simulink model "Hexapod_PD"  (R2026a)
settings: Solver=daessc  StopTime=ref.t(end)  FixedStep=2e-5
InitFcn:
  | startup
model workspace: external: MATLAB File Hexapod_DataFile.m (data not in the file)
undefined symbols (not defined in the file or in its folder): ref, robot, smiData, vc, X, Y, Z
libraries: sm_lib x805, nesl_utility x43
(part 9 of 15)

== system Hexapod_PD/Spherical Joints/MotorRotor_a_4_RIGID ==
  MotorRotor_1_RIGID : Subsystem
  ReferenceFrame : sm_lib/Frames and Transforms/Reference Frame
  ServoArm_1_RIGID : Subsystem
  Transform : sm_lib/Frames and Transforms/Rigid Transform  RotationMethod=ArbitraryAxis  FollAlignAxisA=+X  BaseAlignAxisA=+Y  FollAlignAxisB=+Y  BaseAlignAxisB=+Z  RotationStandardAxis=+Z  RotationAngle=smiData.RigidTransform(22).angle  RotationAngleUnits=rad  RotationArbitraryAxis=smiData.RigidTransform(22).axis  RotationSequenceAxes=FollowerAxes  RotationSequence=XYX  RotationSequenceAngles=[0 0 0]  RotationSequenceAnglesUnits=deg  RotationMatrix=[1 0 0;0 1 0;0 0 1]  Quaternion=[1 0 0 0]  TranslationMethod=Cartesian  TranslationCartesianOffset=smiData.RigidTransform(22).translation  TranslationCartesianOffsetUnits=mm  TranslationStandardAxis=+Z  TranslationStandardOffset=0  TranslationStandardOffsetUnits=m  TranslationROffset=0  TranslationROffsetUnits=m  TranslationThetaOffset=0  TranslationThetaOffsetUnits=deg  TranslationZOffset=0  TranslationZOffsetUnits=m
  Transform1 : sm_lib/Frames and Transforms/Rigid Transform  RotationMethod=ArbitraryAxis  FollAlignAxisA=+X  BaseAlignAxisA=+Y  FollAlignAxisB=+Y  BaseAlignAxisB=+Z  RotationStandardAxis=+Z  RotationAngle=smiData.RigidTransform(23).angle  RotationAngleUnits=rad  RotationArbitraryAxis=smiData.RigidTransform(23).axis  RotationSequenceAxes=FollowerAxes  RotationSequence=XYX  RotationSequenceAngles=[0 0 0]  RotationSequenceAnglesUnits=deg  RotationMatrix=[1 0 0;0 1 0;0 0 1]  Quaternion=[1 0 0 0]  TranslationMethod=Cartesian  TranslationCartesianOffset=smiData.RigidTransform(23).translation  TranslationCartesianOffsetUnits=mm  TranslationStandardAxis=+Z  TranslationStandardOffset=0  TranslationStandardOffsetUnits=m  TranslationROffset=0  TranslationROffsetUnits=m  TranslationThetaOffset=0  TranslationThetaOffsetUnits=deg  TranslationZOffset=0  TranslationZOffsetUnits=m
  Transform10 : sm_lib/Frames and Transforms/Rigid Transform  RotationMethod=ArbitraryAxis  FollAlignAxisA=+X  BaseAlignAxisA=+Y  FollAlignAxisB=+Y  BaseAlignAxisB=+Z  RotationStandardAxis=+Z  RotationAngle=smiData.RigidTransform(269).angle  RotationAngleUnits=rad  RotationArbitraryAxis=smiData.RigidTransform(269).axis  RotationSequenceAxes=FollowerAxes  RotationSequence=XYX  RotationSequenceAngles=[0 0 0]  RotationSequenceAnglesUnits=deg  RotationMatrix=[1 0 0;0 1 0;0 0 1]  Quaternion=[1 0 0 0]  TranslationMethod=Cartesian  TranslationCartesianOffset=smiData.RigidTransform(269).translation  TranslationCartesianOffsetUnits=mm  TranslationStandardAxis=+Z  TranslationStandardOffset=0  TranslationStandardOffsetUnits=m  TranslationROffset=0  TranslationROffsetUnits=m  TranslationThetaOffset=0  TranslationThetaOffsetUnits=deg  TranslationZOffset=0  TranslationZOffsetUnits=m
  Transform11 : sm_lib/Frames and Transforms/Rigid Transform  RotationMethod=ArbitraryAxis  FollAlignAxisA=+X  BaseAlignAxisA=+Y  FollAlignAxisB=+Y  BaseAlignAxisB=+Z  RotationStandardAxis=+Z  RotationAngle=smiData.RigidTransform(270).angle  RotationAngleUnits=rad  RotationArbitraryAxis=smiData.RigidTransform(270).axis  RotationSequenceAxes=FollowerAxes  RotationSequence=XYX  RotationSequenceAngles=[0 0 0]  RotationSequenceAnglesUnits=deg  RotationMatrix=[1 0 0;0 1 0;0 0 1]  Quaternion=[1 0 0 0]  TranslationMethod=Cartesian  TranslationCartesianOffset=smiData.RigidTransform(270).translation  TranslationCartesianOffsetUnits=mm  TranslationStandardAxis=+Z  TranslationStandardOffset=0  TranslationStandardOffsetUnits=m  TranslationROffset=0  TranslationROffsetUnits=m  TranslationThetaOffset=0  TranslationThetaOffsetUnits=deg  TranslationZOffset=0  TranslationZOffsetUnits=m
  Transform2 : sm_lib/Frames and Transforms/Rigid Transform  RotationMethod=ArbitraryAxis  FollAlignAxisA=+X  BaseAlignAxisA=+Y  FollAlignAxisB=+Y  BaseAlignAxisB=+Z  RotationStandardAxis=+Z  RotationAngle=smiData.RigidTransform(261).angle  RotationAngleUnits=rad  RotationArbitraryAxis=smiData.RigidTransform(261).axis  RotationSequenceAxes=FollowerAxes  RotationSequence=XYX  RotationSequenceAngles=[0 0 0]  RotationSequenceAnglesUnits=deg  RotationMatrix=[1 0 0;0 1 0;0 0 1]  Quaternion=[1 0 0 0]  TranslationMethod=Cartesian  TranslationCartesianOffset=smiData.RigidTransform(261).translation  TranslationCartesianOffsetUnits=mm  TranslationStandardAxis=+Z  TranslationStandardOffset=0  TranslationStandardOffsetUnits=m  TranslationROffset=0  TranslationROffsetUnits=m  TranslationThetaOffset=0  TranslationThetaOffsetUnits=deg  TranslationZOffset=0  TranslationZOffsetUnits=m
  Transform3 : sm_lib/Frames and Transforms/Rigid Transform  RotationMethod=ArbitraryAxis  FollAlignAxisA=+X  BaseAlignAxisA=+Y  FollAlignAxisB=+Y  BaseAlignAxisB=+Z  RotationStandardAxis=+Z  RotationAngle=smiData.RigidTransform(262).angle  RotationAngleUnits=rad  RotationArbitraryAxis=smiData.RigidTransform(262).axis  RotationSequenceAxes=FollowerAxes  RotationSequence=XYX  RotationSequenceAngles=[0 0 0]  RotationSequenceAnglesUnits=deg  RotationMatrix=[1 0 0;0 1 0;0 0 1]  Quaternion=[1 0 0 0]  TranslationMethod=Cartesian  TranslationCartesianOffset=smiData.RigidTransform(262).translation  TranslationCartesianOffsetUnits=mm  TranslationStandardAxis=+Z  TranslationStandardOffset=0  TranslationStandardOffsetUnits=m  TranslationROffset=0  TranslationROffsetUnits=m  TranslationThetaOffset=0  TranslationThetaOffsetUnits=deg  TranslationZOffset=0  TranslationZOffsetUnits=m
  Transform4 : sm_lib/Frames and Transforms/Rigid Transform  RotationMethod=ArbitraryAxis  FollAlignAxisA=+X  BaseAlignAxisA=+Y  FollAlignAxisB=+Y  BaseAlignAxisB=+Z  RotationStandardAxis=+Z  RotationAngle=smiData.RigidTransform(263).angle  RotationAngleUnits=rad  RotationArbitraryAxis=smiData.RigidTransform(263).axis  RotationSequenceAxes=FollowerAxes  RotationSequence=XYX  RotationSequenceAngles=[0 0 0]  RotationSequenceAnglesUnits=deg  RotationMatrix=[1 0 0;0 1 0;0 0 1]  Quaternion=[1 0 0 0]  TranslationMethod=Cartesian  TranslationCartesianOffset=smiData.RigidTransform(263).translation  TranslationCartesianOffsetUnits=mm  TranslationStandardAxis=+Z  TranslationStandardOffset=0  TranslationStandardOffsetUnits=m  TranslationROffset=0  TranslationROffsetUnits=m  TranslationThetaOffset=0  TranslationThetaOffsetUnits=deg  TranslationZOffset=0  TranslationZOffsetUnits=m
  Transform5 : sm_lib/Frames and Transforms/Rigid Transform  RotationMethod=ArbitraryAxis  FollAlignAxisA=+X  BaseAlignAxisA=+Y  FollAlignAxisB=+Y  BaseAlignAxisB=+Z  RotationStandardAxis=+Z  RotationAngle=smiData.RigidTransform(264).angle  RotationAngleUnits=rad  RotationArbitraryAxis=smiData.RigidTransform(264).axis  RotationSequenceAxes=FollowerAxes  RotationSequence=XYX  RotationSequenceAngles=[0 0 0]  RotationSequenceAnglesUnits=deg  RotationMatrix=[1 0 0;0 1 0;0 0 1]  Quaternion=[1 0 0 0]  TranslationMethod=Cartesian  TranslationCartesianOffset=smiData.RigidTransform(264).translation  TranslationCartesianOffsetUnits=mm  TranslationStandardAxis=+Z  TranslationStandardOffset=0  TranslationStandardOffsetUnits=m  TranslationROffset=0  TranslationROffsetUnits=m  TranslationThetaOffset=0  TranslationThetaOffsetUnits=deg  TranslationZOffset=0  TranslationZOffsetUnits=m
  Transform6 : sm_lib/Frames and Transforms/Rigid Transform  RotationMethod=ArbitraryAxis  FollAlignAxisA=+X  BaseAlignAxisA=+Y  FollAlignAxisB=+Y  BaseAlignAxisB=+Z  RotationStandardAxis=+Z  RotationAngle=smiData.RigidTransform(265).angle  RotationAngleUnits=rad  RotationArbitraryAxis=smiData.RigidTransform(265).axis  RotationSequenceAxes=FollowerAxes  RotationSequence=XYX  RotationSequenceAngles=[0 0 0]  RotationSequenceAnglesUnits=deg  RotationMatrix=[1 0 0;0 1 0;0 0 1]  Quaternion=[1 0 0 0]  TranslationMethod=Cartesian  TranslationCartesianOffset=smiData.RigidTransform(265).translation  TranslationCartesianOffsetUnits=mm  TranslationStandardAxis=+Z  TranslationStandardOffset=0  TranslationStandardOffsetUnits=m  TranslationROffset=0  TranslationROffsetUnits=m  TranslationThetaOffset=0  TranslationThetaOffsetUnits=deg  TranslationZOffset=0  TranslationZOffsetUnits=m
  Transform7 : sm_lib/Frames and Transforms/Rigid Transform  RotationMethod=ArbitraryAxis  FollAlignAxisA=+X  BaseAlignAxisA=+Y  FollAlignAxisB=+Y  BaseAlignAxisB=+Z  RotationStandardAxis=+Z  RotationAngle=smiData.RigidTransform(266).angle  RotationAngleUnits=rad  RotationArbitraryAxis=smiData.RigidTransform(266).axis  RotationSequenceAxes=FollowerAxes  RotationSequence=XYX  RotationSequenceAngles=[0 0 0]  RotationSequenceAnglesUnits=deg  RotationMatrix=[1 0 0;0 1 0;0 0 1]  Quaternion=[1 0 0 0]  TranslationMethod=Cartesian  TranslationCartesianOffset=smiData.RigidTransform(266).translation  TranslationCartesianOffsetUnits=mm  TranslationStandardAxis=+Z  TranslationStandardOffset=0  TranslationStandardOffsetUnits=m  TranslationROffset=0  TranslationROffsetUnits=m  TranslationThetaOffset=0  TranslationThetaOffsetUnits=deg  TranslationZOffset=0  TranslationZOffsetUnits=m
  Transform8 : sm_lib/Frames and Transforms/Rigid Transform  RotationMethod=ArbitraryAxis  FollAlignAxisA=+X  BaseAlignAxisA=+Y  FollAlignAxisB=+Y  BaseAlignAxisB=+Z  RotationStandardAxis=+Z  RotationAngle=smiData.RigidTransform(267).angle  RotationAngleUnits=rad  RotationArbitraryAxis=smiData.RigidTransform(267).axis  RotationSequenceAxes=FollowerAxes  RotationSequence=XYX  RotationSequenceAngles=[0 0 0]  RotationSequenceAnglesUnits=deg  RotationMatrix=[1 0 0;0 1 0;0 0 1]  Quaternion=[1 0 0 0]  TranslationMethod=Cartesian  TranslationCartesianOffset=smiData.RigidTransform(267).translation  TranslationCartesianOffsetUnits=mm  TranslationStandardAxis=+Z  TranslationStandardOffset=0  TranslationStandardOffsetUnits=m  TranslationROffset=0  TranslationROffsetUnits=m  TranslationThetaOffset=0  TranslationThetaOffsetUnits=deg  TranslationZOffset=0  TranslationZOffsetUnits=m
  Transform9 : sm_lib/Frames and Transforms/Rigid Transform  RotationMethod=ArbitraryAxis  FollAlignAxisA=+X  BaseAlignAxisA=+Y  FollAlignAxisB=+Y  BaseAlignAxisB=+Z  RotationStandardAxis=+Z  RotationAngle=smiData.RigidTransform(268).angle  RotationAngleUnits=rad  RotationArbitraryAxis=smiData.RigidTransform(268).axis  RotationSequenceAxes=FollowerAxes  RotationSequence=XYX  RotationSequenceAngles=[0 0 0]  RotationSequenceAnglesUnits=deg  RotationMatrix=[1 0 0;0 1 0;0 0 1]  Quaternion=[1 0 0 0]  TranslationMethod=Cartesian  TranslationCartesianOffset=smiData.RigidTransform(268).translation  TranslationCartesianOffsetUnits=mm  TranslationStandardAxis=+Z  TranslationStandardOffset=0  TranslationStandardOffsetUnits=m  TranslationROffset=0  TranslationROffsetUnits=m  TranslationThetaOffset=0  TranslationThetaOffsetUnits=deg  TranslationZOffset=0  TranslationZOffsetUnits=m
  ball_1_RIGID : Subsystem
  x90790A185_Black_Oxide_Steel_High_Heavy_Profile_Cap_Nut_1_RIGID : Subsystem
  x91259A628_Alloy_Steel_Shoulder_Screw_1_RIGID : Subsystem
  x91273A784_Same_Size_Thread_18_8_Stainless_Steel_Shoulder_Screw_1_RIGID : Subsystem
  x91273A784_Same_Size_Thread_18_8_Stainless_Steel_Shoulder_Screw_2_RIGID : Subsystem
  x91273A784_Same_Size_Thread_18_8_Stainless_Steel_Shoulder_Screw_3_RIGID : Subsystem
  x92510A494_Aluminum_Unthreaded_Spacer_1_RIGID : Subsystem
  x93413A312_Black_Super_Corrosion_Resistant_Coated_Steel_Washer_1_RIGID : Subsystem
  B : PMIOPort  Side=Left
  F : PMIOPort  Port=2  Side=Right
  connections:
  Transform/RConn1 -- B/RConn1
  ReferenceFrame/RConn1 -- Transform11/LConn1 -- Transform6/LConn1 -- Transform4/LConn1 -- Transform/LConn1 -- Transform7/LConn1 -- Transform8/LConn1 -- Transform10/LConn1 -- Transform5/LConn1 -- Transform3/LConn1 -- Transform1/LConn1 -- Transform9/LConn1 -- Transform2/LConn1
  Transform1/RConn1 -- F/RConn1
  Transform3/RConn1 -- x91273A784_Same_Size_Thread_18_8_Stainless_Steel_Shoulder_Screw_2_RIGID/LConn1
  Transform7/RConn1 -- x91259A628_Alloy_Steel_Shoulder_Screw_1_RIGID/LConn1
  Transform10/RConn1 -- x92510A494_Aluminum_Unthreaded_Spacer_1_RIGID/LConn1
  Transform8/RConn1 -- x91273A784_Same_Size_Thread_18_8_Stainless_Steel_Shoulder_Screw_1_RIGID/LConn1
  Transform5/RConn1 -- x93413A312_Black_Super_Corrosion_Resistant_Coated_Steel_Washer_1_RIGID/LConn1
  Transform9/RConn1 -- MotorRotor_1_RIGID/LConn1
  Transform2/RConn1 -- ball_1_RIGID/LConn1
  Transform4/RConn1 -- x90790A185_Black_Oxide_Steel_High_Heavy_Profile_Cap_Nut_1_RIGID/LConn1
  Transform11/RConn1 -- ServoArm_1_RIGID/LConn1
  Transform6/RConn1 -- x91273A784_Same_Size_Thread_18_8_Stainless_Steel_Shoulder_Screw_3_RIGID/LConn1

== system Hexapod_PD/Spherical Joints/MotorRotor_a_5_RIGID ==
  MotorRotor_1_RIGID : Subsystem
  ReferenceFrame : sm_lib/Frames and Transforms/Reference Frame
  ServoArm_1_RIGID : Subsystem
  Transform : sm_lib/Frames and Transforms/Rigid Transform  RotationMethod=ArbitraryAxis  FollAlignAxisA=+X  BaseAlignAxisA=+Y  FollAlignAxisB=+Y  BaseAlignAxisB=+Z  RotationStandardAxis=+Z  RotationAngle=smiData.RigidTransform(10).angle  RotationAngleUnits=rad  RotationArbitraryAxis=smiData.RigidTransform(10).axis  RotationSequenceAxes=FollowerAxes  RotationSequence=XYX  RotationSequenceAngles=[0 0 0]  RotationSequenceAnglesUnits=deg  RotationMatrix=[1 0 0;0 1 0;0 0 1]  Quaternion=[1 0 0 0]  TranslationMethod=Cartesian  TranslationCartesianOffset=smiData.RigidTransform(10).translation  TranslationCartesianOffsetUnits=mm  TranslationStandardAxis=+Z  TranslationStandardOffset=0  TranslationStandardOffsetUnits=m  TranslationROffset=0  TranslationROffsetUnits=m  TranslationThetaOffset=0  TranslationThetaOffsetUnits=deg  TranslationZOffset=0  TranslationZOffsetUnits=m
  Transform1 : sm_lib/Frames and Transforms/Rigid Transform  RotationMethod=ArbitraryAxis  FollAlignAxisA=+X  BaseAlignAxisA=+Y  FollAlignAxisB=+Y  BaseAlignAxisB=+Z  RotationStandardAxis=+Z  RotationAngle=smiData.RigidTransform(11).angle  RotationAngleUnits=rad  RotationArbitraryAxis=smiData.RigidTransform(11).axis  RotationSequenceAxes=FollowerAxes  RotationSequence=XYX  RotationSequenceAngles=[0 0 0]  RotationSequenceAnglesUnits=deg  RotationMatrix=[1 0 0;0 1 0;0 0 1]  Quaternion=[1 0 0 0]  TranslationMethod=Cartesian  TranslationCartesianOffset=smiData.RigidTransform(11).translation  TranslationCartesianOffsetUnits=mm  TranslationStandardAxis=+Z  TranslationStandardOffset=0  TranslationStandardOffsetUnits=m  TranslationROffset=0  TranslationROffsetUnits=m  TranslationThetaOffset=0  TranslationThetaOffsetUnits=deg  TranslationZOffset=0  TranslationZOffsetUnits=m
  Transform10 : sm_lib/Frames and Transforms/Rigid Transform  RotationMethod=ArbitraryAxis  FollAlignAxisA=+X  BaseAlignAxisA=+Y  FollAlignAxisB=+Y  BaseAlignAxisB=+Z  RotationStandardAxis=+Z  RotationAngle=smiData.RigidTransform(279).angle  RotationAngleUnits=rad  RotationArbitraryAxis=smiData.RigidTransform(279).axis  RotationSequenceAxes=FollowerAxes  RotationSequence=XYX  RotationSequenceAngles=[0 0 0]  RotationSequenceAnglesUnits=deg  RotationMatrix=[1 0 0;0 1 0;0 0 1]  Quaternion=[1 0 0 0]  TranslationMethod=Cartesian  TranslationCartesianOffset=smiData.RigidTransform(279).translation  TranslationCartesianOffsetUnits=mm  TranslationStandardAxis=+Z  TranslationStandardOffset=0  TranslationStandardOffsetUnits=m  TranslationROffset=0  TranslationROffsetUnits=m  TranslationThetaOffset=0  TranslationThetaOffsetUnits=deg  TranslationZOffset=0  TranslationZOffsetUnits=m
  Transform11 : sm_lib/Frames and Transforms/Rigid Transform  RotationMethod=ArbitraryAxis  FollAlignAxisA=+X  BaseAlignAxisA=+Y  FollAlignAxisB=+Y  BaseAlignAxisB=+Z  RotationStandardAxis=+Z  RotationAngle=smiData.RigidTransform(280).angle  RotationAngleUnits=rad  RotationArbitraryAxis=smiData.RigidTransform(280).axis  RotationSequenceAxes=FollowerAxes  RotationSequence=XYX  RotationSequenceAngles=[0 0 0]  RotationSequenceAnglesUnits=deg  RotationMatrix=[1 0 0;0 1 0;0 0 1]  Quaternion=[1 0 0 0]  TranslationMethod=Cartesian  TranslationCartesianOffset=smiData.RigidTransform(280).translation  TranslationCartesianOffsetUnits=mm  TranslationStandardAxis=+Z  TranslationStandardOffset=0  TranslationStandardOffsetUnits=m  TranslationROffset=0  TranslationROffsetUnits=m  TranslationThetaOffset=0  TranslationThetaOffsetUnits=deg  TranslationZOffset=0  TranslationZOffsetUnits=m
  Transform2 : sm_lib/Frames and Transforms/Rigid Transform  RotationMethod=ArbitraryAxis  FollAlignAxisA=+X  BaseAlignAxisA=+Y  FollAlignAxisB=+Y  BaseAlignAxisB=+Z  RotationStandardAxis=+Z  RotationAngle=smiData.RigidTransform(271).angle  RotationAngleUnits=rad  RotationArbitraryAxis=smiData.RigidTransform(271).axis  RotationSequenceAxes=FollowerAxes  RotationSequence=XYX  RotationSequenceAngles=[0 0 0]  RotationSequenceAnglesUnits=deg  RotationMatrix=[1 0 0;0 1 0;0 0 1]  Quaternion=[1 0 0 0]  TranslationMethod=Cartesian  TranslationCartesianOffset=smiData.RigidTransform(271).translation  TranslationCartesianOffsetUnits=mm  TranslationStandardAxis=+Z  TranslationStandardOffset=0  TranslationStandardOffsetUnits=m  TranslationROffset=0  TranslationROffsetUnits=m  TranslationThetaOffset=0  TranslationThetaOffsetUnits=deg  TranslationZOffset=0  TranslationZOffsetUnits=m
  Transform3 : sm_lib/Frames and Transforms/Rigid Transform  RotationMethod=ArbitraryAxis  FollAlignAxisA=+X  BaseAlignAxisA=+Y  FollAlignAxisB=+Y  BaseAlignAxisB=+Z  RotationStandardAxis=+Z  RotationAngle=smiData.RigidTransform(272).angle  RotationAngleUnits=rad  RotationArbitraryAxis=smiData.RigidTransform(272).axis  RotationSequenceAxes=FollowerAxes  RotationSequence=XYX  RotationSequenceAngles=[0 0 0]  RotationSequenceAnglesUnits=deg  RotationMatrix=[1 0 0;0 1 0;0 0 1]  Quaternion=[1 0 0 0]  TranslationMethod=Cartesian  TranslationCartesianOffset=smiData.RigidTransform(272).translation  TranslationCartesianOffsetUnits=mm  TranslationStandardAxis=+Z  TranslationStandardOffset=0  TranslationStandardOffsetUnits=m  TranslationROffset=0  TranslationROffsetUnits=m  TranslationThetaOffset=0  TranslationThetaOffsetUnits=deg  TranslationZOffset=0  TranslationZOffsetUnits=m
  Transform4 : sm_lib/Frames and Transforms/Rigid Transform  RotationMethod=ArbitraryAxis  FollAlignAxisA=+X  BaseAlignAxisA=+Y  FollAlignAxisB=+Y  BaseAlignAxisB=+Z  RotationStandardAxis=+Z  RotationAngle=smiData.RigidTransform(273).angle  RotationAngleUnits=rad  RotationArbitraryAxis=smiData.RigidTransform(273).axis  RotationSequenceAxes=FollowerAxes  RotationSequence=XYX  RotationSequenceAngles=[0 0 0]  RotationSequenceAnglesUnits=deg  RotationMatrix=[1 0 0;0 1 0;0 0 1]  Quaternion=[1 0 0 0]  TranslationMethod=Cartesian  TranslationCartesianOffset=smiData.RigidTransform(273).translation  TranslationCartesianOffsetUnits=mm  TranslationStandardAxis=+Z  TranslationStandardOffset=0  TranslationStandardOffsetUnits=m  TranslationROffset=0  TranslationROffsetUnits=m  TranslationThetaOffset=0  TranslationThetaOffsetUnits=deg  TranslationZOffset=0  TranslationZOffsetUnits=m
  Transform5 : sm_lib/Frames and Transforms/Rigid Transform  RotationMethod=ArbitraryAxis  FollAlignAxisA=+X  BaseAlignAxisA=+Y  FollAlignAxisB=+Y  BaseAlignAxisB=+Z  RotationStandardAxis=+Z  RotationAngle=smiData.RigidTransform(274).angle  RotationAngleUnits=rad  RotationArbitraryAxis=smiData.RigidTransform(274).axis  RotationSequenceAxes=FollowerAxes  RotationSequence=XYX  RotationSequenceAngles=[0 0 0]  RotationSequenceAnglesUnits=deg  RotationMatrix=[1 0 0;0 1 0;0 0 1]  Quaternion=[1 0 0 0]  TranslationMethod=Cartesian  TranslationCartesianOffset=smiData.RigidTransform(274).translation  TranslationCartesianOffsetUnits=mm  TranslationStandardAxis=+Z  TranslationStandardOffset=0  TranslationStandardOffsetUnits=m  TranslationROffset=0  TranslationROffsetUnits=m  TranslationThetaOffset=0  TranslationThetaOffsetUnits=deg  TranslationZOffset=0  TranslationZOffsetUnits=m
  Transform6 : sm_lib/Frames and Transforms/Rigid Transform  RotationMethod=ArbitraryAxis  FollAlignAxisA=+X  BaseAlignAxisA=+Y  FollAlignAxisB=+Y  BaseAlignAxisB=+Z  RotationStandardAxis=+Z  RotationAngle=smiData.RigidTransform(275).angle  RotationAngleUnits=rad  RotationArbitraryAxis=smiData.RigidTransform(275).axis  RotationSequenceAxes=FollowerAxes  RotationSequence=XYX  RotationSequenceAngles=[0 0 0]  RotationSequenceAnglesUnits=deg  RotationMatrix=[1 0 0;0 1 0;0 0 1]  Quaternion=[1 0 0 0]  TranslationMethod=Cartesian  TranslationCartesianOffset=smiData.RigidTransform(275).translation  TranslationCartesianOffsetUnits=mm  TranslationStandardAxis=+Z  TranslationStandardOffset=0  TranslationStandardOffsetUnits=m  TranslationROffset=0  TranslationROffsetUnits=m  TranslationThetaOffset=0  TranslationThetaOffsetUnits=deg  TranslationZOffset=0  TranslationZOffsetUnits=m
  Transform7 : sm_lib/Frames and Transforms/Rigid Transform  RotationMethod=ArbitraryAxis  FollAlignAxisA=+X  BaseAlignAxisA=+Y  FollAlignAxisB=+Y  BaseAlignAxisB=+Z  RotationStandardAxis=+Z  RotationAngle=smiData.RigidTransform(276).angle  RotationAngleUnits=rad  RotationArbitraryAxis=smiData.RigidTransform(276).axis  RotationSequenceAxes=FollowerAxes  RotationSequence=XYX  RotationSequenceAngles=[0 0 0]  RotationSequenceAnglesUnits=deg  RotationMatrix=[1 0 0;0 1 0;0 0 1]  Quaternion=[1 0 0 0]  TranslationMethod=Cartesian  TranslationCartesianOffset=smiData.RigidTransform(276).translation  TranslationCartesianOffsetUnits=mm  TranslationStandardAxis=+Z  TranslationStandardOffset=0  TranslationStandardOffsetUnits=m  TranslationROffset=0  TranslationROffsetUnits=m  TranslationThetaOffset=0  TranslationThetaOffsetUnits=deg  TranslationZOffset=0  TranslationZOffsetUnits=m
  Transform8 : sm_lib/Frames and Transforms/Rigid Transform  RotationMethod=ArbitraryAxis  FollAlignAxisA=+X  BaseAlignAxisA=+Y  FollAlignAxisB=+Y  BaseAlignAxisB=+Z  RotationStandardAxis=+Z  RotationAngle=smiData.RigidTransform(277).angle  RotationAngleUnits=rad  RotationArbitraryAxis=smiData.RigidTransform(277).axis  RotationSequenceAxes=FollowerAxes  RotationSequence=XYX  RotationSequenceAngles=[0 0 0]  RotationSequenceAnglesUnits=deg  RotationMatrix=[1 0 0;0 1 0;0 0 1]  Quaternion=[1 0 0 0]  TranslationMethod=Cartesian  TranslationCartesianOffset=smiData.RigidTransform(277).translation  TranslationCartesianOffsetUnits=mm  TranslationStandardAxis=+Z  TranslationStandardOffset=0  TranslationStandardOffsetUnits=m  TranslationROffset=0  TranslationROffsetUnits=m  TranslationThetaOffset=0  TranslationThetaOffsetUnits=deg  TranslationZOffset=0  TranslationZOffsetUnits=m
  Transform9 : sm_lib/Frames and Transforms/Rigid Transform  RotationMethod=ArbitraryAxis  FollAlignAxisA=+X  BaseAlignAxisA=+Y  FollAlignAxisB=+Y  BaseAlignAxisB=+Z  RotationStandardAxis=+Z  RotationAngle=smiData.RigidTransform(278).angle  RotationAngleUnits=rad  RotationArbitraryAxis=smiData.RigidTransform(278).axis  RotationSequenceAxes=FollowerAxes  RotationSequence=XYX  RotationSequenceAngles=[0 0 0]  RotationSequenceAnglesUnits=deg  RotationMatrix=[1 0 0;0 1 0;0 0 1]  Quaternion=[1 0 0 0]  TranslationMethod=Cartesian  TranslationCartesianOffset=smiData.RigidTransform(278).translation  TranslationCartesianOffsetUnits=mm  TranslationStandardAxis=+Z  TranslationStandardOffset=0  TranslationStandardOffsetUnits=m  TranslationROffset=0  TranslationROffsetUnits=m  TranslationThetaOffset=0  TranslationThetaOffsetUnits=deg  TranslationZOffset=0  TranslationZOffsetUnits=m
  ball_1_RIGID : Subsystem
  x90790A185_Black_Oxide_Steel_High_Heavy_Profile_Cap_Nut_1_RIGID : Subsystem
  x91259A628_Alloy_Steel_Shoulder_Screw_1_RIGID : Subsystem
  x91273A784_Same_Size_Thread_18_8_Stainless_Steel_Shoulder_Screw_1_RIGID : Subsystem
  x91273A784_Same_Size_Thread_18_8_Stainless_Steel_Shoulder_Screw_2_RIGID : Subsystem
  x91273A784_Same_Size_Thread_18_8_Stainless_Steel_Shoulder_Screw_3_RIGID : Subsystem
  x92510A494_Aluminum_Unthreaded_Spacer_1_RIGID : Subsystem
  x93413A312_Black_Super_Corrosion_Resistant_Coated_Steel_Washer_1_RIGID : Subsystem
  B : PMIOPort  Side=Left
  F : PMIOPort  Port=2  Side=Right
  connections:
  Transform/LConn1 -- ReferenceFrame/RConn1 -- Transform8/LConn1 -- Transform9/LConn1 -- Transform7/LConn1 -- Transform6/LConn1 -- Transform5/LConn1 -- Transform4/LConn1 -- Transform3/LConn1 -- Transform2/LConn1 -- Transform11/LConn1 -- Transform10/LConn1 -- Transform1/LConn1
  Transform/RConn1 -- B/RConn1
  MotorRotor_1_RIGID/LConn1 -- Transform9/RConn1
  Transform10/RConn1 -- x92510A494_Aluminum_Unthreaded_Spacer_1_RIGID/LConn1
  ServoArm_1_RIGID/LConn1 -- Transform11/RConn1
  Transform1/RConn1 -- F/RConn1
  Transform2/RConn1 -- ball_1_RIGID/LConn1
  Transform3/RConn1 -- x91273A784_Same_Size_Thread_18_8_Stainless_Steel_Shoulder_Screw_2_RIGID/LConn1
  Transform4/RConn1 -- x90790A185_Black_Oxide_Steel_High_Heavy_Profile_Cap_Nut_1_RIGID/LConn1
  Transform5/RConn1 -- x93413A312_Black_Super_Corrosion_Resistant_Coated_Steel_Washer_1_RIGID/LConn1
  Transform6/RConn1 -- x91273A784_Same_Size_Thread_18_8_Stainless_Steel_Shoulder_Screw_3_RIGID/LConn1
  Transform7/RConn1 -- x91259A628_Alloy_Steel_Shoulder_Screw_1_RIGID/LConn1
  Transform8/RConn1 -- x91273A784_Same_Size_Thread_18_8_Stainless_Steel_Shoulder_Screw_1_RIGID/LConn1

== system Hexapod_PD/Spherical Joints/MotorRotor_a_6_RIGID ==
  MotorRotor_1_RIGID : Subsystem
  ReferenceFrame : sm_lib/Frames and Transforms/Reference Frame
  ServoArm_1_RIGID : Subsystem
  Transform : sm_lib/Frames and Transforms/Rigid Transform  RotationMethod=ArbitraryAxis  FollAlignAxisA=+X  BaseAlignAxisA=+Y  FollAlignAxisB=+Y  BaseAlignAxisB=+Z  RotationStandardAxis=+Z  RotationAngle=smiData.RigidTransform(14).angle  RotationAngleUnits=rad  RotationArbitraryAxis=smiData.RigidTransform(14).axis  RotationSequenceAxes=FollowerAxes  RotationSequence=XYX  RotationSequenceAngles=[0 0 0]  RotationSequenceAnglesUnits=deg  RotationMatrix=[1 0 0;0 1 0;0 0 1]  Quaternion=[1 0 0 0]  TranslationMethod=Cartesian  TranslationCartesianOffset=smiData.RigidTransform(14).translation  TranslationCartesianOffsetUnits=mm  TranslationStandardAxis=+Z  TranslationStandardOffset=0  TranslationStandardOffsetUnits=m  TranslationROffset=0  TranslationROffsetUnits=m  TranslationThetaOffset=0  TranslationThetaOffsetUnits=deg  TranslationZOffset=0  TranslationZOffsetUnits=m
  Transform1 : sm_lib/Frames and Transforms/Rigid Transform  RotationMethod=ArbitraryAxis  FollAlignAxisA=+X  BaseAlignAxisA=+Y  FollAlignAxisB=+Y  BaseAlignAxisB=+Z  RotationStandardAxis=+Z  RotationAngle=smiData.RigidTransform(15).angle  RotationAngleUnits=rad  RotationArbitraryAxis=smiData.RigidTransform(15).axis  RotationSequenceAxes=FollowerAxes  RotationSequence=XYX  RotationSequenceAngles=[0 0 0]  RotationSequenceAnglesUnits=deg  RotationMatrix=[1 0 0;0 1 0;0 0 1]  Quaternion=[1 0 0 0]  TranslationMethod=Cartesian  TranslationCartesianOffset=smiData.RigidTransform(15).translation  TranslationCartesianOffsetUnits=mm  TranslationStandardAxis=+Z  TranslationStandardOffset=0  TranslationStandardOffsetUnits=m  TranslationROffset=0  TranslationROffsetUnits=m  TranslationThetaOffset=0  TranslationThetaOffsetUnits=deg  TranslationZOffset=0  TranslationZOffsetUnits=m
  Transform10 : sm_lib/Frames and Transforms/Rigid Transform  RotationMethod=ArbitraryAxis  FollAlignAxisA=+X  BaseAlignAxisA=+Y  FollAlignAxisB=+Y  BaseAlignAxisB=+Z  RotationStandardAxis=+Z  RotationAngle=smiData.RigidTransform(246).angle  RotationAngleUnits=rad  RotationArbitraryAxis=smiData.RigidTransform(246).axis  RotationSequenceAxes=FollowerAxes  RotationSequence=XYX  RotationSequenceAngles=[0 0 0]  RotationSequenceAnglesUnits=deg  RotationMatrix=[1 0 0;0 1 0;0 0 1]  Quaternion=[1 0 0 0]  TranslationMethod=Cartesian  TranslationCartesianOffset=smiData.RigidTransform(246).translation  TranslationCartesianOffsetUnits=mm  TranslationStandardAxis=+Z  TranslationStandardOffset=0  TranslationStandardOffsetUnits=m  TranslationROffset=0  TranslationROffsetUnits=m  TranslationThetaOffset=0  TranslationThetaOffsetUnits=deg  TranslationZOffset=0  TranslationZOffsetUnits=m
  Transform11 : sm_lib/Frames and Transforms/Rigid Transform  RotationMethod=ArbitraryAxis  FollAlignAxisA=+X  BaseAlignAxisA=+Y  FollAlignAxisB=+Y  BaseAlignAxisB=+Z  RotationStandardAxis=+Z  RotationAngle=smiData.RigidTransform(247).angle  RotationAngleUnits=rad  RotationArbitraryAxis=smiData.RigidTransform(247).axis  RotationSequenceAxes=FollowerAxes  RotationSequence=XYX  RotationSequenceAngles=[0 0 0]  RotationSequenceAnglesUnits=deg  RotationMatrix=[1 0 0;0 1 0;0 0 1]  Quaternion=[1 0 0 0]  TranslationMethod=Cartesian  TranslationCartesianOffset=smiData.RigidTransform(247).translation  TranslationCartesianOffsetUnits=mm  TranslationStandardAxis=+Z  TranslationStandardOffset=0  TranslationStandardOffsetUnits=m  TranslationROffset=0  TranslationROffsetUnits=m  TranslationThetaOffset=0  TranslationThetaOffsetUnits=deg  TranslationZOffset=0  TranslationZOffsetUnits=m
  Transform2 : sm_lib/Frames and Transforms/Rigid Transform  RotationMethod=ArbitraryAxis  FollAlignAxisA=+X  BaseAlignAxisA=+Y  FollAlignAxisB=+Y  BaseAlignAxisB=+Z  RotationStandardAxis=+Z  RotationAngle=smiData.RigidTransform(238).angle  RotationAngleUnits=rad  RotationArbitraryAxis=smiData.RigidTransform(238).axis  RotationSequenceAxes=FollowerAxes  RotationSequence=XYX  RotationSequenceAngles=[0 0 0]  RotationSequenceAnglesUnits=deg  RotationMatrix=[1 0 0;0 1 0;0 0 1]  Quaternion=[1 0 0 0]  TranslationMethod=Cartesian  TranslationCartesianOffset=smiData.RigidTransform(238).translation  TranslationCartesianOffsetUnits=mm  TranslationStandardAxis=+Z  TranslationStandardOffset=0  TranslationStandardOffsetUnits=m  TranslationROffset=0  TranslationROffsetUnits=m  TranslationThetaOffset=0  TranslationThetaOffsetUnits=deg  TranslationZOffset=0  TranslationZOffsetUnits=m
  Transform3 : sm_lib/Frames and Transforms/Rigid Transform  RotationMethod=ArbitraryAxis  FollAlignAxisA=+X  BaseAlignAxisA=+Y  FollAlignAxisB=+Y  BaseAlignAxisB=+Z  RotationStandardAxis=+Z  RotationAngle=smiData.RigidTransform(239).angle  RotationAngleUnits=rad  RotationArbitraryAxis=smiData.RigidTransform(239).axis  RotationSequenceAxes=FollowerAxes  RotationSequence=XYX  RotationSequenceAngles=[0 0 0]  RotationSequenceAnglesUnits=deg  RotationMatrix=[1 0 0;0 1 0;0 0 1]  Quaternion=[1 0 0 0]  TranslationMethod=Cartesian  TranslationCartesianOffset=smiData.RigidTransform(239).translation  TranslationCartesianOffsetUnits=mm  TranslationStandardAxis=+Z  TranslationStandardOffset=0  TranslationStandardOffsetUnits=m  TranslationROffset=0  TranslationROffsetUnits=m  TranslationThetaOffset=0  TranslationThetaOffsetUnits=deg  TranslationZOffset=0  TranslationZOffsetUnits=m
  Transform4 : sm_lib/Frames and Transforms/Rigid Transform  RotationMethod=ArbitraryAxis  FollAlignAxisA=+X  BaseAlignAxisA=+Y  FollAlignAxisB=+Y  BaseAlignAxisB=+Z  RotationStandardAxis=+Z  RotationAngle=smiData.RigidTransform(240).angle  RotationAngleUnits=rad  RotationArbitraryAxis=smiData.RigidTransform(240).axis  RotationSequenceAxes=FollowerAxes  RotationSequence=XYX  RotationSequenceAngles=[0 0 0]  RotationSequenceAnglesUnits=deg  RotationMatrix=[1 0 0;0 1 0;0 0 1]  Quaternion=[1 0 0 0]  TranslationMethod=Cartesian  TranslationCartesianOffset=smiData.RigidTransform(240).translation  TranslationCartesianOffsetUnits=mm  TranslationStandardAxis=+Z  TranslationStandardOffset=0  TranslationStandardOffsetUnits=m  TranslationROffset=0  TranslationROffsetUnits=m  TranslationThetaOffset=0  TranslationThetaOffsetUnits=deg  TranslationZOffset=0  TranslationZOffsetUnits=m
  Transform5 : sm_lib/Frames and Transforms/Rigid Transform  RotationMethod=ArbitraryAxis  FollAlignAxisA=+X  BaseAlignAxisA=+Y  FollAlignAxisB=+Y  BaseAlignAxisB=+Z  RotationStandardAxis=+Z  RotationAngle=smiData.RigidTransform(241).angle  RotationAngleUnits=rad  RotationArbitraryAxis=smiData.RigidTransform(241).axis  RotationSequenceAxes=FollowerAxes  RotationSequence=XYX  RotationSequenceAngles=[0 0 0]  RotationSequenceAnglesUnits=deg  RotationMatrix=[1 0 0;0 1 0;0 0 1]  Quaternion=[1 0 0 0]  TranslationMethod=Cartesian  TranslationCartesianOffset=smiData.RigidTransform(241).translation  TranslationCartesianOffsetUnits=mm  TranslationStandardAxis=+Z  TranslationStandardOffset=0  TranslationStandardOffsetUnits=m  TranslationROffset=0  TranslationROffsetUnits=m  TranslationThetaOffset=0  TranslationThetaOffsetUnits=deg  TranslationZOffset=0  TranslationZOffsetUnits=m
  Transform6 : sm_lib/Frames and Transforms/Rigid Transform  RotationMethod=ArbitraryAxis  FollAlignAxisA=+X  BaseAlignAxisA=+Y  FollAlignAxisB=+Y  BaseAlignAxisB=+Z  RotationStandardAxis=+Z  RotationAngle=smiData.RigidTransform(242).angle  RotationAngleUnits=rad  RotationArbitraryAxis=smiData.RigidTransform(242).axis  RotationSequenceAxes=FollowerAxes  RotationSequence=XYX  RotationSequenceAngles=[0 0 0]  RotationSequenceAnglesUnits=deg  RotationMatrix=[1 0 0;0 1 0;0 0 1]  Quaternion=[1 0 0 0]  TranslationMethod=Cartesian  TranslationCartesianOffset=smiData.RigidTransform(242).translation  TranslationCartesianOffsetUnits=mm  TranslationStandardAxis=+Z  TranslationStandardOffset=0  TranslationStandardOffsetUnits=m  TranslationROffset=0  TranslationROffsetUnits=m  TranslationThetaOffset=0  TranslationThetaOffsetUnits=deg  TranslationZOffset=0  TranslationZOffsetUnits=m
  Transform7 : sm_lib/Frames and Transforms/Rigid Transform  RotationMethod=ArbitraryAxis  FollAlignAxisA=+X  BaseAlignAxisA=+Y  FollAlignAxisB=+Y  BaseAlignAxisB=+Z  RotationStandardAxis=+Z  RotationAngle=smiData.RigidTransform(243).angle  RotationAngleUnits=rad  RotationArbitraryAxis=smiData.RigidTransform(243).axis  RotationSequenceAxes=FollowerAxes  RotationSequence=XYX  RotationSequenceAngles=[0 0 0]  RotationSequenceAnglesUnits=deg  RotationMatrix=[1 0 0;0 1 0;0 0 1]  Quaternion=[1 0 0 0]  TranslationMethod=Cartesian  TranslationCartesianOffset=smiData.RigidTransform(243).translation  TranslationCartesianOffsetUnits=mm  TranslationStandardAxis=+Z  TranslationStandardOffset=0  TranslationStandardOffsetUnits=m  TranslationROffset=0  TranslationROffsetUnits=m  TranslationThetaOffset=0  TranslationThetaOffsetUnits=deg  TranslationZOffset=0  TranslationZOffsetUnits=m
  Transform8 : sm_lib/Frames and Transforms/Rigid Transform  RotationMethod=ArbitraryAxis  FollAlignAxisA=+X  BaseAlignAxisA=+Y  FollAlignAxisB=+Y  BaseAlignAxisB=+Z  RotationStandardAxis=+Z  RotationAngle=smiData.RigidTransform(244).angle  RotationAngleUnits=rad  RotationArbitraryAxis=smiData.RigidTransform(244).axis  RotationSequenceAxes=FollowerAxes  RotationSequence=XYX  RotationSequenceAngles=[0 0 0]  RotationSequenceAnglesUnits=deg  RotationMatrix=[1 0 0;0 1 0;0 0 1]  Quaternion=[1 0 0 0]  TranslationMethod=Cartesian  TranslationCartesianOffset=smiData.RigidTransform(244).translation  TranslationCartesianOffsetUnits=mm  TranslationStandardAxis=+Z  TranslationStandardOffset=0  TranslationStandardOffsetUnits=m  TranslationROffset=0  TranslationROffsetUnits=m  TranslationThetaOffset=0  TranslationThetaOffsetUnits=deg  TranslationZOffset=0  TranslationZOffsetUnits=m
  Transform9 : sm_lib/Frames and Transforms/Rigid Transform  RotationMethod=ArbitraryAxis  FollAlignAxisA=+X  BaseAlignAxisA=+Y  FollAlignAxisB=+Y  BaseAlignAxisB=+Z  RotationStandardAxis=+Z  RotationAngle=smiData.RigidTransform(245).angle  RotationAngleUnits=rad  RotationArbitraryAxis=smiData.RigidTransform(245).axis  RotationSequenceAxes=FollowerAxes  RotationSequence=XYX  RotationSequenceAngles=[0 0 0]  RotationSequenceAnglesUnits=deg  RotationMatrix=[1 0 0;0 1 0;0 0 1]  Quaternion=[1 0 0 0]  TranslationMethod=Cartesian  TranslationCartesianOffset=smiData.RigidTransform(245).translation  TranslationCartesianOffsetUnits=mm  TranslationStandardAxis=+Z  TranslationStandardOffset=0  TranslationStandardOffsetUnits=m  TranslationROffset=0  TranslationROffsetUnits=m  TranslationThetaOffset=0  TranslationThetaOffsetUnits=deg  TranslationZOffset=0  TranslationZOffsetUnits=m
  ball_1_RIGID : Subsystem
  x90790A185_Black_Oxide_Steel_High_Heavy_Profile_Cap_Nut_1_RIGID : Subsystem
  x91259A628_Alloy_Steel_Shoulder_Screw_1_RIGID : Subsystem
  x91273A784_Same_Size_Thread_18_8_Stainless_Steel_Shoulder_Screw_1_RIGID : Subsystem
  x91273A784_Same_Size_Thread_18_8_Stainless_Steel_Shoulder_Screw_2_RIGID : Subsystem
  x91273A784_Same_Size_Thread_18_8_Stainless_Steel_Shoulder_Screw_3_RIGID : Subsystem
  x92510A494_Aluminum_Unthreaded_Spacer_1_RIGID : Subsystem
  x93413A312_Black_Super_Corrosion_Resistant_Coated_Steel_Washer_1_RIGID : Subsystem
  B : PMIOPort  Side=Left
  F : PMIOPort  Port=2  Side=Right
  connections:
  Transform/LConn1 -- ReferenceFrame/RConn1 -- Transform8/LConn1 -- Transform9/LConn1 -- Transform7/LConn1 -- Transform6/LConn1 -- Transform5/LConn1 -- Transform4/LConn1 -- Transform3/LConn1 -- Transform2/LConn1 -- Transform11/LConn1 -- Transform10/LConn1 -- Transform1/LConn1
  Transform/RConn1 -- B/RConn1
  MotorRotor_1_RIGID/LConn1 -- Transform9/RConn1
  Transform10/RConn1 -- x92510A494_Aluminum_Unthreaded_Spacer_1_RIGID/LConn1
  ServoArm_1_RIGID/LConn1 -- Transform11/RConn1
  Transform1/RConn1 -- F/RConn1
  Transform2/RConn1 -- ball_1_RIGID/LConn1
  Transform3/RConn1 -- x91273A784_Same_Size_Thread_18_8_Stainless_Steel_Shoulder_Screw_2_RIGID/LConn1
  Transform4/RConn1 -- x90790A185_Black_Oxide_Steel_High_Heavy_Profile_Cap_Nut_1_RIGID/LConn1
  Transform5/RConn1 -- x93413A312_Black_Super_Corrosion_Resistant_Coated_Steel_Washer_1_RIGID/LConn1
  Transform6/RConn1 -- x91273A784_Same_Size_Thread_18_8_Stainless_Steel_Shoulder_Screw_3_RIGID/LConn1
  Transform7/RConn1 -- x91259A628_Alloy_Steel_Shoulder_Screw_1_RIGID/LConn1
  Transform8/RConn1 -- x91273A784_Same_Size_Thread_18_8_Stainless_Steel_Shoulder_Screw_1_RIGID/LConn1

== system Hexapod_PD/Torso pose logger/g ==
  Ina : Inport
  Demux : Demux  Outputs=3
  Mux1 : Mux  Inputs=3
  g : Bias  Bias=robot.g  SaturateOnIntegerOverflow=off
  Outa : Outport
  wires:
  Demux/1 -> Mux1/1
  Demux/3 -> g/1
  Mux1/1 -> Outa/1
  g/1 -> Mux1/3
  Demux/2 -> Mux1/2
  Ina/1 -> Demux/1

== system Hexapod_PD/Base/Base_Side_a_1_RIGID/MotorStator_1_RIGID ==
  ReferenceFrame : sm_lib/Frames and Transforms/Reference Frame
  Solid : sm_lib/Body Elements/File Solid  ExtGeomFileName=MotorStator_Default_sldprt.STEP  UnitType=FromFile  ExtGeomFileUnits=m  StepReaderType=HEX  ExportConvexHullGeometry=off  InertiaType=Custom  BasedOnType=DensityFromFile  Density=1000  DensityUnits=kg/m^3  Mass=smiData.Solid(11).mass  MassUnits=kg  CenterOfMass=smiData.Solid(11).CoM  CenterOfMassUnits=mm  MomentsOfInertia=smiData.Solid(11).MoI  MomentsOfInertiaUnits=kg*mm^2  ProductsOfInertia=smiData.Solid(11).PoI  ProductsOfInertiaUnits=kg*mm^2  GraphicType=FromGeometry  MarkerShape=Sphere  MarkerSize=10  GraphicVisPropType=SimpleVisualProperties  GraphicDiffuseColor=smiData.Solid(11).color  GraphicOpacity=smiData.Solid(11).opacity  GraphicSpecularColor=[0.5 0.5 0.5 1.0]  GraphicAmbientColor=[0.15 0.15 0.15 1.0]  GraphicEmissiveColor=[0.0 0.0 0.0 1.0]  GraphicShininess=75  DoExposeReferenceFrame=on  SerializedFrames=<Frames/>
  F : PMIOPort  Side=Left
  connections:
  Solid/RConn1 -- ReferenceFrame/RConn1 -- F/RConn1

== system Hexapod_PD/Base/Base_Side_a_1_RIGID/MotorStator_2_RIGID ==
  ReferenceFrame : sm_lib/Frames and Transforms/Reference Frame
  Solid : sm_lib/Body Elements/File Solid  ExtGeomFileName=MotorStator_Default_sldprt.STEP  UnitType=FromFile  ExtGeomFileUnits=m  StepReaderType=HEX  ExportConvexHullGeometry=off  InertiaType=Custom  BasedOnType=DensityFromFile  Density=1000  DensityUnits=kg/m^3  Mass=smiData.Solid(11).mass  MassUnits=kg  CenterOfMass=smiData.Solid(11).CoM  CenterOfMassUnits=mm  MomentsOfInertia=smiData.Solid(11).MoI  MomentsOfInertiaUnits=kg*mm^2  ProductsOfInertia=smiData.Solid(11).PoI  ProductsOfInertiaUnits=kg*mm^2  GraphicType=FromGeometry  MarkerShape=Sphere  MarkerSize=10  GraphicVisPropType=SimpleVisualProperties  GraphicDiffuseColor=smiData.Solid(11).color  GraphicOpacity=smiData.Solid(11).opacity  GraphicSpecularColor=[0.5 0.5 0.5 1.0]  GraphicAmbientColor=[0.15 0.15 0.15 1.0]  GraphicEmissiveColor=[0.0 0.0 0.0 1.0]  GraphicShininess=75  DoExposeReferenceFrame=on  SerializedFrames=<Frames/>
  F : PMIOPort  Side=Left
  connections:
  Solid/RConn1 -- ReferenceFrame/RConn1 -- F/RConn1

== system Hexapod_PD/Base/Base_Side_a_1_RIGID/base_plate_corner_connector_mm_1_RIGID ==
  ReferenceFrame : sm_lib/Frames and Transforms/Reference Frame
  Solid : sm_lib/Body Elements/File Solid  ExtGeomFileName=base_plate_corner_connector_mm_Default_sldprt.STEP  UnitType=FromFile  ExtGeomFileUnits=m  StepReaderType=HEX  ExportConvexHullGeometry=off  InertiaType=Custom  BasedOnType=DensityFromFile  Density=1000  DensityUnits=kg/m^3  Mass=smiData.Solid(1).mass  MassUnits=kg  CenterOfMass=smiData.Solid(1).CoM  CenterOfMassUnits=in  MomentsOfInertia=smiData.Solid(1).MoI  MomentsOfInertiaUnits=kg*in^2  ProductsOfInertia=smiData.Solid(1).PoI  ProductsOfInertiaUnits=kg*in^2  GraphicType=FromGeometry  MarkerShape=Sphere  MarkerSize=10  GraphicVisPropType=SimpleVisualProperties  GraphicDiffuseColor=smiData.Solid(1).color  GraphicOpacity=smiData.Solid(1).opacity  GraphicSpecularColor=[0.5 0.5 0.5 1.0]  GraphicAmbientColor=[0.15 0.15 0.15 1.0]  GraphicEmissiveColor=[0.0 0.0 0.0 1.0]  GraphicShininess=75  DoExposeReferenceFrame=on  SerializedFrames=<Frames/>
  F : PMIOPort  Side=Left
  connections:
  Solid/RConn1 -- ReferenceFrame/RConn1 -- F/RConn1

== system Hexapod_PD/Base/Base_Side_a_1_RIGID/base_plate_corner_connector_mm_2_RIGID ==
  ReferenceFrame : sm_lib/Frames and Transforms/Reference Frame
  Solid : sm_lib/Body Elements/File Solid  ExtGeomFileName=base_plate_corner_connector_mm_Default_sldprt.STEP  UnitType=FromFile  ExtGeomFileUnits=m  StepReaderType=HEX  ExportConvexHullGeometry=off  InertiaType=Custom  BasedOnType=DensityFromFile  Density=1000  DensityUnits=kg/m^3  Mass=smiData.Solid(1).mass  MassUnits=kg  CenterOfMass=smiData.Solid(1).CoM  CenterOfMassUnits=in  MomentsOfInertia=smiData.Solid(1).MoI  MomentsOfInertiaUnits=kg*in^2  ProductsOfInertia=smiData.Solid(1).PoI  ProductsOfInertiaUnits=kg*in^2  GraphicType=FromGeometry  MarkerShape=Sphere  MarkerSize=10  GraphicVisPropType=SimpleVisualProperties  GraphicDiffuseColor=smiData.Solid(1).color  GraphicOpacity=smiData.Solid(1).opacity  GraphicSpecularColor=[0.5 0.5 0.5 1.0]  GraphicAmbientColor=[0.15 0.15 0.15 1.0]  GraphicEmissiveColor=[0.0 0.0 0.0 1.0]  GraphicShininess=75  DoExposeReferenceFrame=on  SerializedFrames=<Frames/>
  F : PMIOPort  Side=Left
  connections:
  Solid/RConn1 -- ReferenceFrame/RConn1 -- F/RConn1

== system Hexapod_PD/Base/Base_Side_a_1_RIGID/base_plate_mm_1_RIGID ==
  ReferenceFrame : sm_lib/Frames and Transforms/Reference Frame
  Solid : sm_lib/Body Elements/File Solid  ExtGeomFileName=base_plate_mm_Default_sldprt.STEP  UnitType=FromFile  ExtGeomFileUnits=m  StepReaderType=HEX  ExportConvexHullGeometry=off  InertiaType=Custom  BasedOnType=DensityFromFile  Density=1000  DensityUnits=kg/m^3  Mass=smiData.Solid(8).mass  MassUnits=kg  CenterOfMass=smiData.Solid(8).CoM  CenterOfMassUnits=mm  MomentsOfInertia=smiData.Solid(8).MoI  MomentsOfInertiaUnits=kg*mm^2  ProductsOfInertia=smiData.Solid(8).PoI  ProductsOfInertiaUnits=kg*mm^2  GraphicType=FromGeometry  MarkerShape=Sphere  MarkerSize=10  GraphicVisPropType=SimpleVisualProperties  GraphicDiffuseColor=smiData.Solid(8).color  GraphicOpacity=smiData.Solid(8).opacity  GraphicSpecularColor=[0.5 0.5 0.5 1.0]  GraphicAmbientColor=[0.15 0.15 0.15 1.0]  GraphicEmissiveColor=[0.0 0.0 0.0 1.0]  GraphicShininess=75  DoExposeReferenceFrame=on  SerializedFrames=<Frames/>
  F : PMIOPort  Side=Left
  connections:
  Solid/RConn1 -- ReferenceFrame/RConn1 -- F/RConn1

== system Hexapod_PD/Base/Base_Side_a_1_RIGID/bumper_1_RIGID ==
  ReferenceFrame : sm_lib/Frames and Transforms/Reference Frame
  Solid : sm_lib/Body Elements/File Solid  ExtGeomFileName=bumper_Default_sldprt.STEP  UnitType=FromFile  ExtGeomFileUnits=m  StepReaderType=HEX  ExportConvexHullGeometry=off  InertiaType=Custom  BasedOnType=DensityFromFile  Density=1000  DensityUnits=kg/m^3  Mass=smiData.Solid(7).mass  MassUnits=kg  CenterOfMass=smiData.Solid(7).CoM  CenterOfMassUnits=mm  MomentsOfInertia=smiData.Solid(7).MoI  MomentsOfInertiaUnits=kg*mm^2  ProductsOfInertia=smiData.Solid(7).PoI  ProductsOfInertiaUnits=kg*mm^2  GraphicType=FromGeometry  MarkerShape=Sphere  MarkerSize=10  GraphicVisPropType=SimpleVisualProperties  GraphicDiffuseColor=smiData.Solid(7).color  GraphicOpacity=smiData.Solid(7).opacity  GraphicSpecularColor=[0.5 0.5 0.5 1.0]  GraphicAmbientColor=[0.15 0.15 0.15 1.0]  GraphicEmissiveColor=[0.0 0.0 0.0 1.0]  GraphicShininess=75  DoExposeReferenceFrame=on  SerializedFrames=<Frames/>
  F : PMIOPort  Side=Left
  connections:
  Solid/RConn1 -- ReferenceFrame/RConn1 -- F/RConn1

== system Hexapod_PD/Base/Base_Side_a_1_RIGID/prox_sensor_1_RIGID ==
  ReferenceFrame : sm_lib/Frames and Transforms/Reference Frame
  Solid : sm_lib/Body Elements/File Solid  ExtGeomFileName=prox_sensor_95245A233_sldprt.STEP  UnitType=FromFile  ExtGeomFileUnits=m  StepReaderType=HEX  ExportConvexHullGeometry=off  InertiaType=Custom  BasedOnType=DensityFromFile  Density=1000  DensityUnits=kg/m^3  Mass=smiData.Solid(9).mass  MassUnits=kg  CenterOfMass=smiData.Solid(9).CoM  CenterOfMassUnits=mm  MomentsOfInertia=smiData.Solid(9).MoI  MomentsOfInertiaUnits=kg*mm^2  ProductsOfInertia=smiData.Solid(9).PoI  ProductsOfInertiaUnits=kg*mm^2  GraphicType=FromGeometry  MarkerShape=Sphere  MarkerSize=10  GraphicVisPropType=SimpleVisualProperties  GraphicDiffuseColor=smiData.Solid(9).color  GraphicOpacity=smiData.Solid(9).opacity  GraphicSpecularColor=[0.5 0.5 0.5 1.0]  GraphicAmbientColor=[0.15 0.15 0.15 1.0]  GraphicEmissiveColor=[0.0 0.0 0.0 1.0]  GraphicShininess=75  DoExposeReferenceFrame=on  SerializedFrames=<Frames/>
  F : PMIOPort  Side=Left
  connections:
  Solid/RConn1 -- ReferenceFrame/RConn1 -- F/RConn1

== system Hexapod_PD/Base/Base_Side_a_1_RIGID/prox_sensor_2_RIGID ==
  ReferenceFrame : sm_lib/Frames and Transforms/Reference Frame
  Solid : sm_lib/Body Elements/File Solid  ExtGeomFileName=prox_sensor_95245A233_sldprt.STEP  UnitType=FromFile  ExtGeomFileUnits=m  StepReaderType=HEX  ExportConvexHullGeometry=off  InertiaType=Custom  BasedOnType=DensityFromFile  Density=1000  DensityUnits=kg/m^3  Mass=smiData.Solid(9).mass  MassUnits=kg  CenterOfMass=smiData.Solid(9).CoM  CenterOfMassUnits=mm  MomentsOfInertia=smiData.Solid(9).MoI  MomentsOfInertiaUnits=kg*mm^2  ProductsOfInertia=smiData.Solid(9).PoI  ProductsOfInertiaUnits=kg*mm^2  GraphicType=FromGeometry  MarkerShape=Sphere  MarkerSize=10  GraphicVisPropType=SimpleVisualProperties  GraphicDiffuseColor=smiData.Solid(9).color  GraphicOpacity=smiData.Solid(9).opacity  GraphicSpecularColor=[0.5 0.5 0.5 1.0]  GraphicAmbientColor=[0.15 0.15 0.15 1.0]  GraphicEmissiveColor=[0.0 0.0 0.0 1.0]  GraphicShininess=75  DoExposeReferenceFrame=on  SerializedFrames=<Frames/>
  F : PMIOPort  Side=Left
  connections:
  Solid/RConn1 -- ReferenceFrame/RConn1 -- F/RConn1

== system Hexapod_PD/Base/Base_Side_a_1_RIGID/spacer_1_RIGID ==
  ReferenceFrame : sm_lib/Frames and Transforms/Reference Frame
  Solid : sm_lib/Body Elements/File Solid  ExtGeomFileName=spacer_Default_sldprt.STEP  UnitType=FromFile  ExtGeomFileUnits=m  StepReaderType=HEX  ExportConvexHullGeometry=off  InertiaType=Custom  BasedOnType=DensityFromFile  Density=1000  DensityUnits=kg/m^3  Mass=smiData.Solid(3).mass  MassUnits=kg  CenterOfMass=smiData.Solid(3).CoM  CenterOfMassUnits=mm  MomentsOfInertia=smiData.Solid(3).MoI  MomentsOfInertiaUnits=kg*mm^2  ProductsOfInertia=smiData.Solid(3).PoI  ProductsOfInertiaUnits=kg*mm^2  GraphicType=FromGeometry  MarkerShape=Sphere  MarkerSize=10  GraphicVisPropType=SimpleVisualProperties  GraphicDiffuseColor=smiData.Solid(3).color  GraphicOpacity=smiData.Solid(3).opacity  GraphicSpecularColor=[0.5 0.5 0.5 1.0]  GraphicAmbientColor=[0.15 0.15 0.15 1.0]  GraphicEmissiveColor=[0.0 0.0 0.0 1.0]  GraphicShininess=75  DoExposeReferenceFrame=on  SerializedFrames=<Frames/>
  F : PMIOPort  Side=Left
  connections:
  Solid/RConn1 -- ReferenceFrame/RConn1 -- F/RConn1

== system Hexapod_PD/Base/Base_Side_a_1_RIGID/spacer_2_RIGID ==
  ReferenceFrame : sm_lib/Frames and Transforms/Reference Frame
  Solid : sm_lib/Body Elements/File Solid  ExtGeomFileName=spacer_Default_sldprt.STEP  UnitType=FromFile  ExtGeomFileUnits=m  StepReaderType=HEX  ExportConvexHullGeometry=off  InertiaType=Custom  BasedOnType=DensityFromFile  Density=1000  DensityUnits=kg/m^3  Mass=smiData.Solid(3).mass  MassUnits=kg  CenterOfMass=smiData.Solid(3).CoM  CenterOfMassUnits=mm  MomentsOfInertia=smiData.Solid(3).MoI  MomentsOfInertiaUnits=kg*mm^2  ProductsOfInertia=smiData.Solid(3).PoI  ProductsOfInertiaUnits=kg*mm^2  GraphicType=FromGeometry  MarkerShape=Sphere  MarkerSize=10  GraphicVisPropType=SimpleVisualProperties  GraphicDiffuseColor=smiData.Solid(3).color  GraphicOpacity=smiData.Solid(3).opacity  GraphicSpecularColor=[0.5 0.5 0.5 1.0]  GraphicAmbientColor=[0.15 0.15 0.15 1.0]  GraphicEmissiveColor=[0.0 0.0 0.0 1.0]  GraphicShininess=75  DoExposeReferenceFrame=on  SerializedFrames=<Frames/>
  F : PMIOPort  Side=Left
  connections:
  Solid/RConn1 -- ReferenceFrame/RConn1 -- F/RConn1
